simulink model "lab1_2"  (R2023b)
settings: Solver=VariableStepAuto  StartTime=0.0  StopTime=10.0  RelTol=1e-3
libraries: commdigbbndpm3 x2, commchan3 x1, commrandsrc3 x1
settings Model: Creator=chang  LastModifiedBy=chang

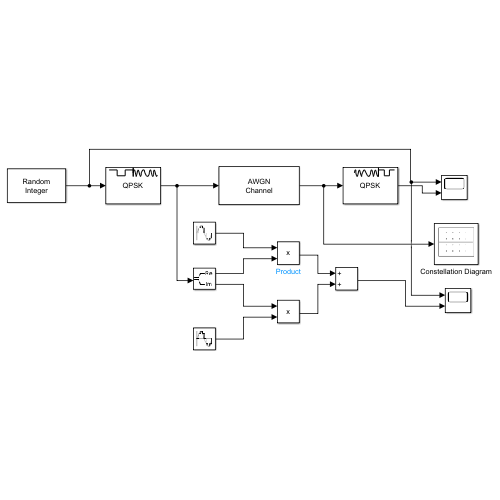
[thumbnail: Simulink's stored preview of the top-level diagram]
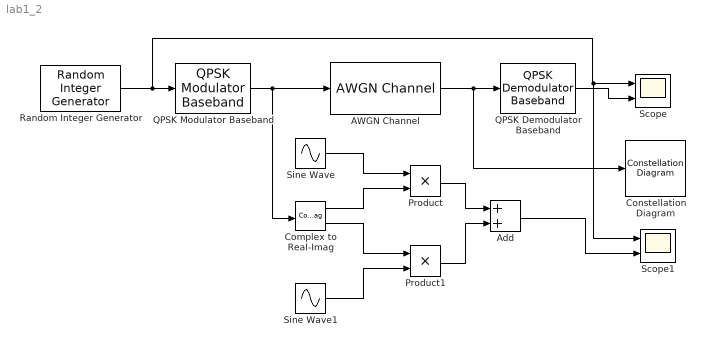
== system lab1_2 ==
  AWGN Channel : commchan3/AWGN Channel  LegacyMode=off  NoiseMethod="Signal to noise ratio  (SNR)"  noiseMode="Signal to noise ratio  (SNR)"  EbNo=10  EsNo=10  SNR=10  BitsPerSymbol=1  SignalPower=2  SamplesPerSymbol=1  SymbolPeriod=1  VarianceSource=Parameter  Variance=1  RandomStream=Global stream  Seed=67  SimulateUsing=Code generation
  Add : Sum
  Complex to Real-Imag : ComplexToRealImag
  Constellation Diagram : ConstellationDiagram  WindowPosition=[1319.000000,190.000000,600.000000,600.000000,]  ScopeFrameLocation=window  SymbolsToDisplaySource=Property  SymbolsToDisplay=1000  XLimits=[-1.46,1.46]  YLimits=[-1.38,1.38]
  Product : Product
  Product1 : Product
  QPSK Demodulator Baseband : commdigbbndpm3/QPSK Demodulator Baseband  OutType=Integer  DecType=Hard decision  VarSource=Dialog  Variance=1  Dec=Gray  Ph=pi/4  outDtype1=Inherit via internal rule  outDtype2=Inherit via internal rule  derotateFactorWordLen=16  derotateFactorDataTypeStr=Inherit: Same word length as input  derotateFactorLastDataTypeStr=Inherit: Same word length as input
  QPSK Modulator Baseband : commdigbbndpm3/QPSK Modulator Baseband  InType=Integer  Enc=Gray  Ph=pi/4  outDtype=double  outWordLen=16  outUDDataType=sfix(16)  outFracLenMode=Best precision  outFracLen=15  outDataTypeStr=double  outLastDataTypeStr=double
  Random Integer Generator : commrandsrc3/Random Integer Generator  SetSize=4  SeedSource=Auto  Seed=0  SampleTime=1  SamplesPerFrame=1  OutputDataType=double  SimulateUsing=Interpreted execution
  Scope : Scope  NumInputPorts=2
  Scope1 : Scope  NumInputPorts=2
  Sine Wave : Sin  Frequency=8*pi  SampleTime=0.001
  Sine Wave1 : Sin  Frequency=8*pi  Phase=pi/2  SampleTime=0.001
  wires:
  QPSK Modulator Baseband/1 -> Complex to Real-Imag/1, AWGN Channel/1
  AWGN Channel/1 -> Constellation Diagram/1, QPSK Demodulator Baseband/1
  QPSK Demodulator Baseband/1 -> Scope/2
  Random Integer Generator/1 -> QPSK Modulator Baseband/1, Scope1/1, Scope/1
  Sine Wave/1 -> Product/1
  Complex to Real-Imag/1 -> Product/2
  Complex to Real-Imag/2 -> Product1/1
  Sine Wave1/1 -> Product1/2
  Product/1 -> Add/1
  Product1/1 -> Add/2
  Add/1 -> Scope1/2
